simulink model "q_aero2_2dof_pp"  (R2024b)
settings: Solver=ode1  StartTime=0.0  StopTime=60  FixedStep=0.002  RelTol=1e-3  EnableMultiTasking=on
values from neighbouring files (symbols this model uses):
  K = place(A, B, desired_poles)    [aero2_2dof_control_pp.m]
undefined symbols (not defined in the file or in its folder): HIL, qc_get_step_size
libraries: quarc_library x6, simulink_extras x4
settings Model: SimulationMode=external  ExtModeTrigDuration=15000  Creator=MLevis  LastModifiedBy=dinhck
settings SolverCC: AlgebraicLoopSolver=TrustRegion  PositivePriorityOrder=on
settings DataIOCC: LimitDataPoints=on  SaveFormat=Array  ReturnWorkspaceOutputs=off
settings DebuggingCC: SolverPrmCheckMsg=warning  UnconnectedInputMsg=warning  UnconnectedOutputMsg=warning  UnconnectedLineMsg=warning  SFUnexpectedBacktrackingDiag=warning  SFNoUnconditionalDefaultTransitionDiag=warning  SFExecutionAtInitializationDiag=none  ArithmeticOperatorsInVariantConditions=warning
settings ModelReferenceCC: EnableRefExpFcnMdlSchedulingChecks=on  PropagateSignalLabelsOutOfModel=off
settings SFSimCC: SimUseLocalCustomCode=off  CustomCodeUndefinedFunction=UseInterfaceOnly
settings RTWCC: Description=QUARC Win64 Target Using Toolchain  SystemTargetFile=quarc_win64.tlc  TemplateMakefile=quarc_default_tmf  RTWUseLocalCustomCode=off  Toolchain=QUARC win64 | nmake (64-bit Windows)  BuildConfiguration=Faster Runs  GPUComputeCapability=3.5  DLArmComputeVersion=19.05
settings CodeAppCC: StateflowObjectComments=on
settings STFCustomTargetCC: ConcurrentExecutionCompliant=on  GRTInterface=on  UseToolchainInfoCompliant=on  SystemTargetFile=quarc_win64.tlc
settings GRTTargetCC: TargetLangStandard=C89/C90 (ANSI)  ParMdlRefBuildCompliant=off  CompOptLevelCompliant=off  CombineOutputUpdateFcns=off  MatFileLogging=off  CPPClassGenCompliant=off  GRTInterface=on  ExtMode=on  ExtModeMexFile=quarc_comm
settings ConfigComp: CovMetricSettings=dw  CovSaveCumulativeToWorkspaceVar=on  CovSaveSingleToWorkspaceVar=on  CovExternalEMLEnable=off  CovSFcnEnable=off

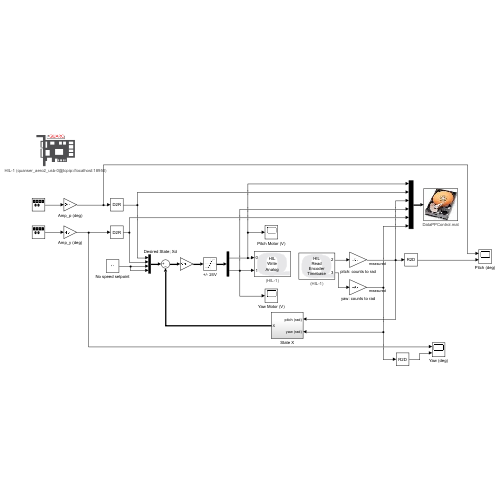
[thumbnail: Simulink's stored preview of the top-level diagram]
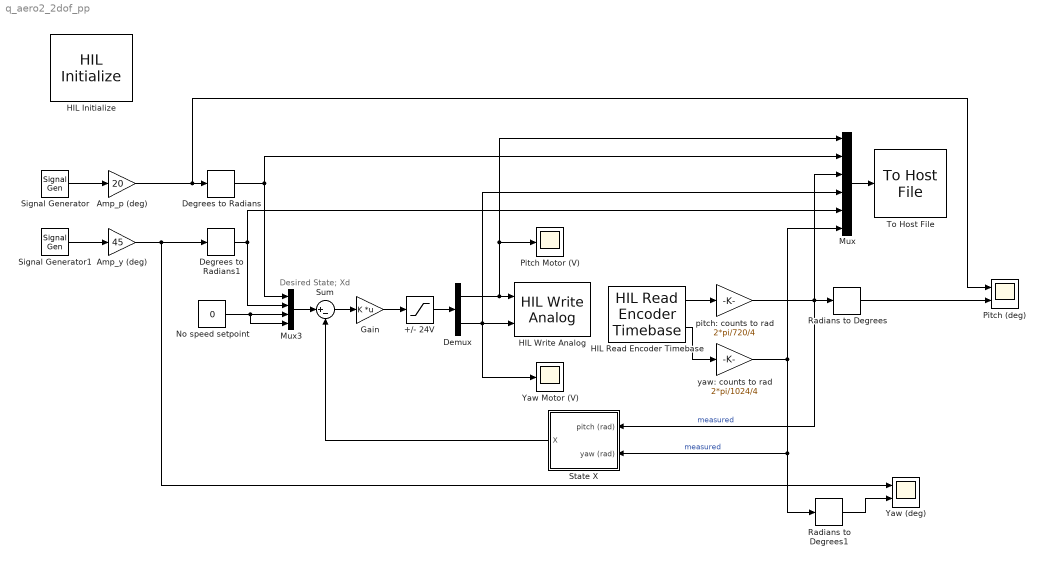
== system q_aero2_2dof_pp ==
  note: Desired State; Xd
  +/- 24V : Saturate  UpperLimit=24  LowerLimit=-24
  Amp_p (deg) : Gain  Gain=20
  Amp_y (deg) : Gain  Gain=45
  Degrees to Radians : simulink_extras/Transformations/Degrees to Radians
  Degrees to Radians1 : simulink_extras/Transformations/Degrees to Radians
  Demux : Demux  Outputs=2
  Gain : Gain  Gain=K  Multiplication=Matrix(K*u)
  HIL Initialize : quarc_library/Data Acquisition/Generic/Configuration/HIL Initialize  Priority=-99  object_name=HIL-1  board_type=quanser_aero2_usb  board_number=0@tcpip://localhost:18950  board_options=""  exclusive=off  active=off  hardware_clocks=[0]  clock_modes=[]  initial_clock_frequencies=[]  set_clock_params_at_start=off  set_clock_params_at_switch_in=off  set_clock_frequencies_at_start=off  set_clock_frequencies_at_switch_in=off  analog_input_channels=[0:1]  analog_input_configurations=[]  analog_input_maximums=3  analog_input_minimums=-3  set_analog_input_params_at_start=off  set_analog_input_params_at_switch_in=off  analog_output_channels=[0:1]  analog_output_maximums=24  analog_output_minimums=-24  initial_analog_outputs=[0]  final_analog_outputs=[0]  watchdog_analog_outputs=[0]  set_analog_output_params_at_start=off  set_analog_output_params_at_switch_in=off  set_analog_outputs_at_start=on  set_analog_outputs_at_switch_in=off  set_analog_outputs_at_terminate=on  set_analog_outputs_at_switch_out=off  set_analog_outputs_on_watchdog=on  digital_input_channels=[]  digital_output_channels=[0:1]  digital_output_configuration=[]  initial_digital_outputs=[1]  final_digital_outputs=[0]  watchdog_digital_outputs=[0]  set_digital_output_params_at_start=off  set_digital_output_params_at_switch_in=off  set_digital_outputs_at_start=on  set_digital_outputs_at_switch_in=off  set_digital_outputs_at_terminate=on  set_digital_outputs_at_switch_out=off  set_digital_outputs_on_watchdog=on  encoder_channels=[0:3]  quadrature=[4]  encoder_filter_frequency=[]  initial_encoder_counts=[0]  set_encoder_params_at_start=off  set_encoder_params_at_switch_in=off  set_encoder_counts_at_start=on  set_encoder_counts_at_switch_in=off  pwm_channels=[]  pwm_modes=[]  pwm_frequency=[]  pwm_configuration=[]  pwm_alignment=[]  pwm_polarity=[]  pwm_leading_deadband=[]  pwm_trailing_deadband=[]  initial_pwm_outputs=[]  final_pwm_outputs=[]  watchdog_pwm_outputs=[]  set_pwm_params_at_start=off  set_pwm_params_at_switch_in=off  set_pwm_outputs_at_start=off  set_pwm_outputs_at_switch_in=off  set_pwm_outputs_at_terminate=off  set_pwm_outputs_at_switch_out=off  set_pwm_outputs_on_watchdog=off  other_output_channels=[11000:11002]  initial_other_outputs=[0 1 0]  final_other_outputs=[1 0 0]  watchdog_other_outputs=[0 0 1]  set_other_outputs_at_start=on  set_other_outputs_at_switch_in=off  set_other_outputs_at_terminate=on  set_other_outputs_at_switch_out=off  set_other_outputs_on_watchdog=on
  HIL Read Encoder Timebase : quarc_library/Data Acquisition/Generic/Timebases/HIL Read Encoder Timebase  object_name=HIL-1  clock=0  channels=[2,3]  active=on  vector_output=off  data_type_mode=Inherit via back propagation  data_type=double  overflow_mode=Error on overflow  samples_in_buffer=max(ceil(1/qc_get_step_size), 1)
  HIL Write Analog : quarc_library/Data Acquisition/Generic/Immediate I//O/HIL Write Analog  object_name=HIL-1  channels=[0:1]  sample_time=-1  active=off  vector_input=off
  Mux : Mux  Inputs=6
  Mux3 : Mux
  No speed setpoint : Constant  Value=0
  Pitch (deg) : Scope  NumInputPorts=2
  Pitch Motor (V) : Scope
  Radians to Degrees : simulink_extras/Transformations/Radians to Degrees
  Radians to Degrees1 : simulink_extras/Transformations/Radians to Degrees
  Signal Generator : SignalGenerator  WaveForm=square  Frequency=0.05
  Signal Generator1 : SignalGenerator  WaveForm=square  Frequency=0.04
  State X : Subsystem
  Sum : Sum  Inputs=|+-
  To Host File : quarc_library/Sinks/To Host/To Host File  source=Specify via dialog (do not evaluate)  file_name=DataPPControl.mat  variable_name=DataPPControl  decimation=1  sample_time=-1  file_format=MAT-file v.4  options=No header or footer  append=off  final_file_name=DataPPControl.mat  bitrate=2000000
  Yaw (deg) : Scope  NumInputPorts=2
  Yaw Motor (V) : Scope
  pitch: counts to rad : Gain  Gain=2*pi/720/4
  yaw: counts to rad : Gain  Gain=2*pi/1024/4
  wires:
  Degrees to Radians/1 -> Mux3/1, Mux/2
  Degrees to Radians1/1 -> Mux/5, Mux3/2
  Signal Generator/1 -> Amp_p (deg)/1
  Amp_p (deg)/1 -> Pitch (deg)/1, Degrees to Radians/1
  Signal Generator1/1 -> Amp_y (deg)/1
  Amp_y (deg)/1 -> Degrees to Radians1/1, Yaw (deg)/1
  Gain/1 -> +/- 24V/1
  Sum/1 -> Gain/1
  Mux3/1 -> Sum/1
  No speed setpoint/1 -> Mux3/4, Mux3/3
  State X/1(X) -> Sum/2
  HIL Read Encoder Timebase/2 -> yaw: counts to rad/1
  HIL Read Encoder Timebase/1 -> pitch: counts to rad/1
  pitch: counts to rad/1 -> Mux/3, Radians to Degrees/1, State X/1(pitch (rad))  "measured"
  yaw: counts to rad/1 -> Mux/6, Radians to Degrees1/1, State X/2(yaw (rad))  "measured"
  +/- 24V/1 -> Demux/1
  Demux/1 -> HIL Write Analog/1, Mux/1, Pitch Motor (V)/1
  Demux/2 -> Yaw Motor (V)/1, Mux/4, HIL Write Analog/2
  Radians to Degrees/1 -> Pitch (deg)/2
  Radians to Degrees1/1 -> Yaw (deg)/2
  Mux/1 -> To Host File/1

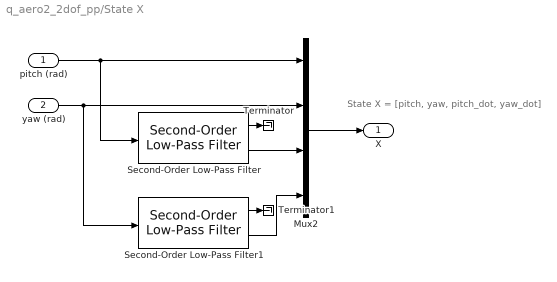
== system q_aero2_2dof_pp/State X ==
  note: State X = [pitch, yaw, pitch_dot, yaw_dot]
  pitch (rad) : Inport
  yaw (rad) : Inport  Port=2
  Mux2 : Mux
  Second-Order Low-Pass Filter : quarc_library/Continuous/Second-Order Low-Pass Filter  params_source=Internal (dialog parameters)  input_width=50  input_zeta=0.8  input_init=0
  Second-Order Low-Pass Filter1 : quarc_library/Continuous/Second-Order Low-Pass Filter  params_source=Internal (dialog parameters)  input_width=50  input_zeta=0.8  input_init=0
  Terminator : Terminator
  Terminator1 : Terminator
  X : Outport
  wires:
  Mux2/1 -> X/1
  yaw (rad)/1 -> Second-Order Low-Pass Filter1/1, Mux2/2
  pitch (rad)/1 -> Second-Order Low-Pass Filter/1, Mux2/1
  Second-Order Low-Pass Filter/2 -> Mux2/3
  Second-Order Low-Pass Filter1/2 -> Mux2/4
  Second-Order Low-Pass Filter/1 -> Terminator/1
  Second-Order Low-Pass Filter1/1 -> Terminator1/1
